simulink model "Lab4_14102026"  (R2019a)
settings: Solver=VariableStepAuto  StartTime=0.0  StopTime=1  RelTol=1e-3  EnableMultiTasking=on
settings Model: Creator=CSE  LastModifiedBy=Admin
settings DataIOCC: ReturnWorkspaceOutputs=off
settings OptimizationCC: LifeSpan=inf
settings DebuggingCC: SFUnexpectedBacktrackingDiag=warning  SFNoUnconditionalDefaultTransitionDiag=warning  ArithmeticOperatorsInVariantConditions=warning
settings SFSimCC: SimUseLocalCustomCode=off
settings RTWCC: RTWUseLocalCustomCode=off
settings CodeAppCC: StateflowObjectComments=on
settings GRTTargetCC: TargetLangStandard=C89/C90 (ANSI)  GeneratePreprocessorConditionals=Disable all
settings ConfigComp: CovMetricSettings=dw  CovHtmlReporting=on  CovSaveCumulativeToWorkspaceVar=on  CovSaveSingleToWorkspaceVar=on  CovExternalEMLEnable=off

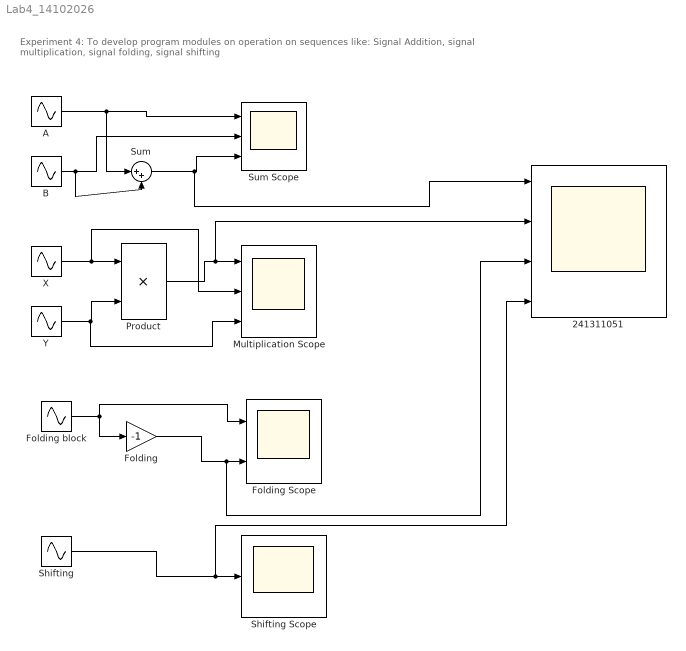
== system Lab4_14102026 ==
  note: Experiment 4: To develop program modules on operation on sequences like: Signal Addition, signal multiplication, signal folding, signal shifting
  241311051 : Scope  NumInputPorts=4
  A : Sin  Amplitude=2  Frequency=2*pi*5  SampleTime=1e-4
  B : Sin  Frequency=2*pi*10  SampleTime=1e-4
  Folding : Gain  Gain=-1
  Folding Scope : Scope  NumInputPorts=2
  "Folding block " : Sin  Frequency=2*pi*10  SampleTime=1e-4
  Multiplication Scope : Scope  NumInputPorts=3
  Product : Product
  Shifting : Sin  Frequency=2*pi*10  Phase=-1  SampleTime=1e-4
  Shifting Scope : Scope
  Sum : Sum  Inputs=|++
  Sum Scope : Scope  NumInputPorts=3
  X : Sin  Amplitude=2  Frequency=2*pi*5  SampleTime=1e-4
  Y : Sin  Frequency=2*pi*10  SampleTime=1e-4
  wires:
  A/1 -> Sum/1, Sum Scope/1
  B/1 -> Sum/2, Sum Scope/2
  Sum/1 -> 241311051/1, Sum Scope/3
  X/1 -> Multiplication Scope/2, Product/1
  Y/1 -> Multiplication Scope/3, Product/2
  Product/1 -> 241311051/2, Multiplication Scope/1
  "Folding block "/1 -> Folding Scope/1, Folding/1
  Folding/1 -> 241311051/3, Folding Scope/2
  Shifting/1 -> 241311051/4, Shifting Scope/1
